simulink model "ArduCopter_TemplateController"  (R2018b)
settings: Solver=FixedStepDiscrete  StartTime=0.0  StopTime=1000  FixedStep=1/400  RelTol=1e-4
libraries: ardupilot_custom_controller_lib x2
settings Model: DataTypeOverride=Single  DataTypeOverrideAppliesTo=Floating-point  Creator=Yannic  LastModifiedBy=yannic
settings SolverCC: ZeroCrossControl=DisableAll
settings DataIOCC: LimitDataPoints=on  SaveOutput=off  SaveTime=off  ReturnWorkspaceOutputs=on
settings OptimizationCC: DefaultParameterBehavior=Inlined  UseFloatMulNetSlope=on  DefaultUnderspecifiedDataType=single  InlineInvariantSignals=on  PassReuseOutputArgsAs=Individual arguments  ZeroExternalMemoryAtStartup=off  ZeroInternalMemoryAtStartup=off  NoFixptDivByZeroProtection=on  EfficientFloat2IntCast=on  LifeSpan=1  OptimizeBlockOrder=speed  DifferentSizesBufferReuse=on
settings DebuggingCC: ReadBeforeWriteMsg=DisableAll  WriteAfterWriteMsg=DisableAll  WriteAfterReadMsg=DisableAll  MultiTaskDSMMsg=none  ParameterTunabilityLossMsg=error  AllowSymbolicDim=off  LibraryContextMissingDiagnostic=none  SFUnexpectedBacktrackingDiag=warning  SFNoUnconditionalDefaultTransitionDiag=warning  SFExecutionAtInitializationDiag=none
settings HardwareCC: ProdBitPerLong=64  ProdLongLongMode=on  ProdHWDeviceType=Intel->x86-64 (Linux 64)
settings ModelReferenceCC: UpdateModelReferenceTargets=IfOutOfDate  PropagateSignalLabelsOutOfModel=off
settings SFSimCC: SFSimEcho=off  SimUseLocalCustomCode=off  MATLABDynamicMemAlloc=off
settings RTWCC: SystemTargetFile=ert.tlc  GenCodeOnly=on  TemplateMakefile=ert_default_tmf  GenerateReport=on  RTWUseLocalCustomCode=off  IncludeHyperlinkInReport=on  LaunchReport=on  TargetLang=C++  GenerateTraceInfo=on  GenerateTraceReport=on  GenerateTraceReportSl=on  GenerateTraceReportSf=on  GenerateTraceReportEml=on
settings CodeAppCC: ForceParamTrailComments=on  IgnoreCustomStorageClasses=off  OperatorAnnotations=on  SimulinkDataObjDesc=on  SFDataObjDesc=on  CustomSymbolStrGlobalVar=rt$N$M  CustomSymbolStrType=$N$M  CustomSymbolStrFcn=$N$M$F  CustomSymbolStrMacro=$N$M  InsertBlockDesc=on
settings ERTTargetCC: TargetLangStandard=C++03 (ISO)  GenerateSampleERTMain=on  IncludeMdlTerminateFcn=off  CombineSignalStateStructs=on  SuppressErrorStatus=on  SupportAbsoluteTime=off  MultiInstanceERTCode=on  CodeInterfacePackaging=C++ class  SupportNonFinite=off  SupportComplex=off  ERTHeaderFileRootName=MatlabController$E  ERTSourceFileRootName=MatlabController$E  ERTDataFileRootName=MatlabController_data  InlinedParameterPlacement=NonHierarchical  RootIOFormat=Structure reference  ERTCustomFileTemplate=example_file_process.tlc  ERTFilePackagingFormat=CompactWithDataFile
settings ConfigComp: CovMetricSettings=dw  CovHtmlReporting=on  CovSaveCumulativeToWorkspaceVar=on  CovSaveSingleToWorkspaceVar=on  CovExternalEMLEnable=off

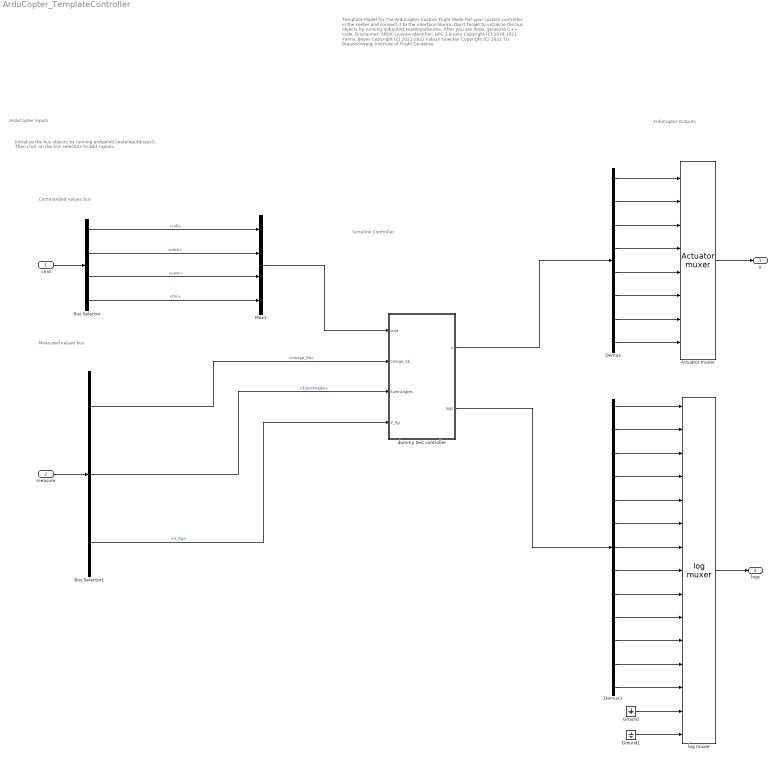
== system ArduCopter_TemplateController ==
  note: Measured values bus
  note: Initialize the bus objects by running ardupilotCreateInputBuses().
      | Then click on the bus selectors to add signals.
  note: Commanded values bus
  note: ArduCopter Inputs
  note: ArduCopter Outputs
  note: Simulink Controller
  note: Template Model for The ArduCopter Custom Flight Mode
      |
      | Put your custom controller in the center and connect it to the interface blocks.
      | Don't forget to initialize the bus objects by running ardupilotCreateInputBuses.
      | After you are done, generate C++ code.
      |
      | Disclaimer:
      | SPDX-License-Identifier: GPL-3.0-only
      |
      | Copyright (C) 2019-2021 Yannic Beyer
      | Copyright (C) 2021-2022 Fabian Guecker
      | Copyright (C) 2022 TU Braunschweig, Institute of Flight Guidance
  cmd : Inport  OutDataTypeStr=Bus: cmdBus
  measure : Inport  Port=2  OutDataTypeStr=Bus: measureBus
  Actuator muxer : ardupilot_custom_controller_lib/Actuator muxer
      settings: SourceProductName=LADAC
  Bus Selector : BusSelector  OutputSignals=roll,pitch,yaw,thr
  Bus Selector1 : BusSelector  OutputSignals=omega_Kb,EulerAngles,V_Kg
  Demux : Demux  Outputs=8
  Demux1 : Demux  Outputs=13
  Ground : Ground
  Ground1 : Ground
  Mux1 : Mux
  dummy test controller : Subsystem
  log muxer : ardupilot_custom_controller_lib/log muxer  batch_name_1='ML1'  num_signals_1=14  batch_name_2='ML2'  num_signals_2=1  batch_name_3='ML3'  num_signals_3=0  batch_name_4='ML4'  num_signals_4=0  batch_name_5='ML5'  num_signals_5=0
      settings: SourceProductName=LADAC
  u : Outport
  logs : Outport  Port=2
  wires:
  cmd/1 -> Bus Selector/1
  measure/1 -> Bus Selector1/1
  Bus Selector1/2 -> dummy test controller/3(EulerAngles)  "<EulerAngles>"
  Bus Selector1/1 -> dummy test controller/2(omega_Kb)  "<omega_Kb>"
  Bus Selector/1 -> Mux1/1  "<roll>"
  Bus Selector/2 -> Mux1/2  "<pitch>"
  Bus Selector/3 -> Mux1/3  "<yaw>"
  Bus Selector/4 -> Mux1/4  "<thr>"
  Mux1/1 -> dummy test controller/1(cmd)
  dummy test controller/1(u) -> Demux/1
  Actuator muxer/1 -> u/1
  Bus Selector1/3 -> dummy test controller/4(V_Kg)  "<V_Kg>"
  log muxer/1 -> logs/1
  Demux/8 -> Actuator muxer/8
  Demux/7 -> Actuator muxer/7
  Demux/6 -> Actuator muxer/6
  Demux/5 -> Actuator muxer/5
  Demux/4 -> Actuator muxer/4
  Demux/3 -> Actuator muxer/3
  Demux/2 -> Actuator muxer/2
  Demux/1 -> Actuator muxer/1
  Demux1/1 -> log muxer/1
  Demux1/2 -> log muxer/2
  Demux1/3 -> log muxer/3
  Demux1/4 -> log muxer/4
  Demux1/5 -> log muxer/5
  Demux1/6 -> log muxer/6
  Demux1/7 -> log muxer/7
  Demux1/8 -> log muxer/8
  Demux1/9 -> log muxer/9
  Demux1/10 -> log muxer/10
  Demux1/11 -> log muxer/11
  Demux1/12 -> log muxer/12
  Demux1/13 -> log muxer/13
  dummy test controller/2(logs) -> Demux1/1
  Ground/1 -> log muxer/14
  Ground1/1 -> log muxer/15

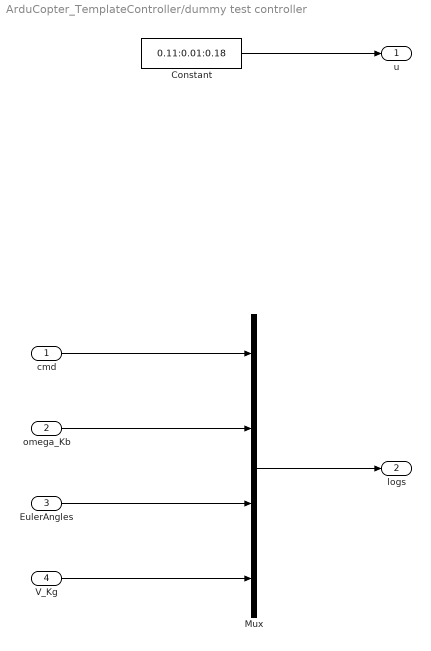
== system ArduCopter_TemplateController/dummy test controller ==
  cmd : Inport
  omega_Kb : Inport  Port=2
  EulerAngles : Inport  Port=3
  V_Kg : Inport  Port=4
  Constant : Constant  Value=0.11:0.01:0.18
  Mux : Mux
  u : Outport
  logs : Outport  Port=2
  wires:
  Constant/1 -> u/1
  Mux/1 -> logs/1
  omega_Kb/1 -> Mux/2
  cmd/1 -> Mux/1
  EulerAngles/1 -> Mux/3
  V_Kg/1 -> Mux/4
